simulink model "reduce_emf_simple"  (R2024b)
settings: Solver=FixedStepAuto  StartTime=0.0  StopTime=25  FixedStep=Tsim  RelTol=1e-4  EnableMultiTasking=on
InitFcn:
  | clc;
  | clear;
  | %% Parameters of the motor
  | Tsim = 1e-6;
  | Tpwm=1e-4;
  | Ts = 1e-4;
  | R = 1.8665;
  | Rs=1.8665;
  | Ls=8.96e-3;
  | Ld = 8.96e-3;
  | Lq = 8.96e-3;
  | L1=(Ld +Lq )/2;
  | L2=(Lq -Ld )/2;
  | flux = 0.21;
  | F=0.00008;
  | J=0.003;
  | Np=4;
  | fpwm = 10e3;
  | Vdc=311;
  | wn=100;
  | %% Controller limiter                                                           % Maximum torque (Nm)
  | I_max = 7.5;                                                    % Maximum current (A)
  | V_max = Vdc/sqrt(3);
  | 
  | 
  | %% 转速环电流环带宽
  | wspd=20;
  | wcur=500;
  | 
  | %% LESO
  | w0=10000;
  | beta1=2*w0-R/Ld;
  | beta2=w0*w0;
  | %% IF启动
  | Iq_if=7;
  | we_if_acc=300;
  | we_if_max=180;
  | we_switch=150;
model workspace (MAT data in the model file):
  new = 0
undefined symbols (not defined in the file or in its folder): DiscIntNeverNeededParam
libraries: spsDCVoltageSourceLib x1, spsGroundLib x1, spsPermanentMagnetSynchronousMachineLib x1, spsUniversalBridgeLib x1, spspowerguiLib x1, simulink x1
(part 2 of 2)

== matlab function reduce_emf_simple/参数辨识与采集/参数辨识算法/参数辨识 ==
  settings: updateMethod=DISCRETE  sampleTime=1e-4
  data: ud input; uq input; id input; iq input; we input; stage input; Ls output size=1; psi output size=1; Rs output size=1; da output size=1; db output size=1; doneL output size=1; doneR output size=1; run output size=1; n output size=1; ack output size=1; R0 output size=1; V0 output size=1
function [Ls, psi, Rs, da, db, doneL, doneR, run, n, ack, R0, V0] = ...
    fcn(ud, uq, id, iq, we, stage)
%#codegen
% ud、uq：V；id、iq：A；we：电角速度rad/s；采样周期Ts=100us。
% Ls：H；psi：Wb；Rs：欧姆；da、db：两组位置误差rad。
% stage=2/3/4为A组基准/正注入/负注入，6/7/8为B组，9为计算。
% run=0等待，1采样，2计算角度，3递推，30完成；负数表示数据缺失。
% n为实际递推次数，ack为采样完成的阶段号；未计算的参数为NaN。
stage = double(stage);

% 六段数据均按[ud uq id iq we]存储，每段取最后2000拍。
persistent dq_data dq_mean ready stage_z tick stopped
% 一电周期滑动平均。
persistent dq_buf dq_sum pos count N
% 跨阶段连续积分，用于修正角度计算中的电阻和逆变器压降。
persistent theta we_z ab_z int_ab int_data has_prev
% 正负注入差：电压/转速、电流/转速、电流、压降系数/转速。
persistent dU dU_w dI_w dI dV_w H F pre
% 辨识结果及RLS状态。x=[Ls/0.01; psi/0.2]仅做数值尺度归一化。
persistent L flux R delta done status ack_z loss x P it

%% 1. 初始化与阶段切换
if isempty(stage_z)
    stage_z = -1;
end
if isempty(dq_data) || ((stage == 0 || stage == 2) && stage ~= stage_z)
    dq_data = zeros(2000, 5, 6);
    dq_mean = zeros(6, 5);
    ready = false(6, 1);
    stopped = false;
    tick = 0;
    dq_buf = zeros(1257, 5);
    dq_sum = zeros(1, 5);
    pos = 0;
    count = 0;
    N = 1;
    theta = 0;
    we_z = 0;
    ab_z = zeros(1, 6);
    int_ab = zeros(1, 6);
    int_data = zeros(2000, 8, 2);
    has_prev = false;
    dU = zeros(2, 2);
    dU_w = zeros(2, 2);
    dI_w = zeros(2, 2);
    dI = zeros(2, 2);
    dV_w = zeros(2, 2);
    H = zeros(3, 3, 2);
    F = zeros(3, 6, 2);
    pre = 0;
    L = NaN;
    flux = NaN;
    R = NaN;
    delta = zeros(2, 1);
    done = zeros(2, 1);
    status = 0;
    ack_z = 0;
    loss = [NaN; NaN];
    x = zeros(2, 1);
    P = 10*eye(2);
    it = 0;
end

dq = [ud uq id iq we];
valid = all(isfinite(dq)) && isfinite(stage);
if valid && stage ~= stage_z
    stage_z = stage;
    tick = 0;
    ack_z = 0;
    dq_buf(:) = 0;
    dq_sum(:) = 0;
    pos = 0;
    count = 0;
    N = 1;
end

if ~valid
    % 非有限输入才中止；不按纹波大小或参数正负拒绝结果。
    L = NaN;
    flux = NaN;
    R = NaN;
    delta(:) = 0;
    done(:) = 0;
    loss(:) = NaN;
    ready(:) = false;
    it = 0;
    status = -1;
    ack_z = 0;
    if stage >= 2 && stage <= 8
        ack_z = -double(stage);
    end
    stopped = true;
end

%% 2. 采样：先等待0.4秒，再保存0.2秒
if ~stopped && stage >= 2 && stage <= 8
    % 积分使用外部50Hz低通后的dq量，阶段5也连续积分。
    % 它只用于压降修正，不改变控制环角度或转速。
    if has_prev
        theta = mod(theta + 0.5e-4*(we_z + we), 2*pi);
    end
    c = cos(theta);
    s = sin(theta);
    ab = [ud*c-uq*s, ud*s+uq*c, id*c-iq*s, id*s+iq*c];
    D = (4/pi)*ab(3:4)/max(hypot(id, iq), 1e-12);
    ab_now = [ab D];
    if has_prev
        int_ab = int_ab + 0.5e-4*(ab_z + ab_now);
    end
    ab_z = ab_now;
    we_z = we;
    has_prev = true;

    % A组对应存储段1~3，B组对应存储段4~6，阶段5留给恢复。
    seg = 0;
    if stage >= 2 && stage <= 4
        seg = double(stage) - 1;
    elseif stage >= 6 && stage <= 8
        seg = double(stage) - 2;
    end

    if seg > 0 && ~ready(seg)
        status = 1;
        tick = tick + 1;
        % 0.1秒时锁定周期点数；五路量使用完全相同的平均器。
        if tick == 1000
            N = min(1257, max(50, round(2*pi/(max(abs(we), 50)*1e-4))));
            dq_buf(:) = 0;
            dq_sum(:) = 0;
            pos = 0;
            count = 0;
        end
        dq_avg = dq;
        if tick >= 1000
            pos = mod(pos, N) + 1;
            dq_sum = dq_sum + dq - dq_buf(pos, :);
            dq_buf(pos, :) = dq;
            count = min(N, count + 1);
            dq_avg = dq_sum/count;
        end
        if tick > 4000 && tick <= 6000
            k = tick - 4000;
            dq_data(k, :, seg) = dq_avg;
            if seg == 1 || seg == 4
                g = 1 + (seg == 4);
                int_data(k, :, g) = [int_ab c s];
            end
        end
        if tick == 6000
            dq_mean(seg, :) = sum(dq_data(:, :, seg), 1)/2000;
            ready(seg) = true;
            ack_z = double(stage);
        end
    end
end

%% 3. 正负注入求角度，两组数据交替做参数递推
if ~stopped && stage == 9
    if ~all(ready)
        status = -2;
        stopped = true;
    elseif status == 1
        status = 2;
    elseif pre < 400
        % 每拍处理5个新样本；400拍处理完每组2000个注入样本。
        pre = pre + 1;
        for g = 1:2
            seg = 2 + 3*(g-1);
            for k = (pre-1)*5+1:pre*5
                dq_p = dq_data(k, :, seg);
                dq_m = dq_data(k, :, seg+1);
                wp = speed_safe(dq_p(5));
                wm = speed_safe(dq_m(5));
                Dp = (4/pi)*dq_p(3:4)/max(hypot(dq_p(3), dq_p(4)), 1e-12);
                Dm = (4/pi)*dq_m(3:4)/max(hypot(dq_m(3), dq_m(4)), 1e-12);
                dU(g, :) = dU(g, :) + dq_p(1:2) - dq_m(1:2);
                dU_w(g, :) = dU_w(g, :) + (dq_p(1:2)/wp - dq_m(1:2)/wm);
                dI_w(g, :) = dI_w(g, :) + (dq_p(3:4)/wp - dq_m(3:4)/wm);
                dI(g, :) = dI(g, :) + (dq_p(3:4) - dq_m(3:4));
                dV_w(g, :) = dV_w(g, :) + (Dp/wp - Dm/wm);
                h = [1; int_data(k, 7, g); int_data(k, 8, g)];
                H(:, :, g) = H(:, :, g) + h*h';
                F(:, :, g) = F(:, :, g) + h*int_data(k, 1:6, g);
            end
            delta(g) = angle_wrap(atan2(dU(g, 2), dU(g, 1)));
        end
        if pre == 400
            loss = loss_fit(H, F);
            for g = 1:2
                delta(g) = angle_fix(dU_w(g, :), dI_w(g, :), ...
                    dI(g, :), dV_w(g, :), loss, 0);
            end
        end
    else
        % A1、B1、A2、B2……每拍读取一个未使用的基准样本。
        it = it + 1;
        for g = 1:2
            delta(g) = angle_fix(dU_w(g, :), dI_w(g, :), ...
                dI(g, :), dV_w(g, :), loss, 0.01*x(1));
        end
        g = 1 + mod(it-1, 2);
        k = floor((it-1)/2) + 1;
        seg = 1 + 3*(g-1);
        ud_k = dq_data(k, 1, seg);
        uq_k = dq_data(k, 2, seg);
        id_k = dq_data(k, 3, seg);
        iq_k = dq_data(k, 4, seg);
        we_k = dq_data(k, 5, seg);

        % 稳态方程消去R：uq*id-ud*iq = we*Ls*(id²+iq²)
        %                                 + we*psi*(id*cos(delta)+iq*sin(delta))。
        phi = [0.01*we_k*(id_k^2+iq_k^2); ...
            0.2*we_k*(id_k*cos(delta(g))+iq_k*sin(delta(g)))];
        scale = max(norm(phi), 1e-12);
        phi = phi/scale;
        u = (uq_k*id_k - ud_k*iq_k)/scale;
        K = P*phi/(1 + phi'*P*phi);
        e = u - phi'*x;
        x = x + K*e;
        % Joseph形式更新协方差，遗忘因子为1。
        A = eye(2) - K*phi';
        P = A*P*A' + K*K';
        P = 0.5*(P + P');
        L = 0.01*x(1);
        flux = 0.2*x(2);
        R = rs_calc(dq_mean, delta, L, flux);
        status = 3;
        if it == 4000
            done(1) = double(all(isfinite(x)));
            done(2) = double(isfinite(R));
            status = 30;
            stopped = true;
        end
    end
end

if ~stopped && stage == 10
    status = -10;
    stopped = true;
end

%% 4. 各电气量独立输出
Ls = L;
psi = flux;
Rs = R;
da = delta(1);
db = delta(2);
doneL = done(1);
doneR = done(2);
run = status;
n = it;
ack = ack_z;
R0 = loss(1);
V0 = loss(2);
end

function a = angle_fix(dU_w, dI_w, dI, dV_w, loss, Ls)
% 正负注入的ud/we、uq/we差分；修正电阻、压降和电流变化的影响。
% R0、V0来自数据标定，Ls来自当前RLS结果，不预填额定参数。
fd = dU_w(1) - loss(1)*dI_w(1) + Ls*dI(2) - loss(2)*dV_w(1);
fq = dU_w(2) - loss(1)*dI_w(2) - Ls*dI(1) - loss(2)*dV_w(2);
a = angle_wrap(atan2(fq, fd));
end

function a = angle_wrap(a)
% 位置误差取论文反正切对应的[-pi/2, pi/2]分支。
if a > pi/2
    a = a - pi;
elseif a < -pi/2
    a = a + pi;
end
end

function loss = loss_fit(H, F)
% 压降修正的辅助计算，不是论文的主参数RLS。
% 将积分量拟合为常值+余弦+正弦，取两个工作点的积分中心差。
% 静止坐标系电压方程给出：DeltaU = R0*DeltaI + V0*DeltaD。
center = zeros(2, 6);
for g = 1:2
    coef = (H(:, :, g) + 1e-10*eye(3))\F(:, :, g);
    center(g, :) = coef(1, :);
end
dInt = center(2, :) - center(1, :);
B = [dInt(3:4)', dInt(5:6)'];
u = dInt(1:2)';
scale = max(sqrt(sum(sum(B.^2))), 1e-12);
B = B/scale;
u = u/scale;
loss = (B'*B + 1e-10*eye(2))\(B'*u);
end

function Rs = rs_calc(dq_mean, delta, Ls, psi)
% 两组q轴方程：uq-we*Ls*id-we*psi*cos(delta) = Rs*iq + V0*Dq。
% 消去共同的V0，每次使用新Ls、psi更新Rs；不直接复制辅助电阻R0。
Dq = zeros(2, 1);
uq_res = zeros(2, 1);
for g = 1:2
    seg = 1 + 3*(g-1);
    id = dq_mean(seg, 3);
    iq = dq_mean(seg, 4);
    we = dq_mean(seg, 5);
    Dq(g) = (4/pi)*iq/max(hypot(id, iq), 1e-8);
    uq_res(g) = dq_mean(seg, 2) - we*Ls*id - we*psi*cos(delta(g));
end
den = Dq(2)*dq_mean(1, 4) - Dq(1)*dq_mean(4, 4);
scale = abs(Dq(2)*dq_mean(1, 4)) + abs(Dq(1)*dq_mean(4, 4));
if abs(den) > 64*eps(max(scale, 1))
    Rs = (Dq(2)*uq_res(1) - Dq(1)*uq_res(2))/den;
else
    Rs = NaN;
end
end

function we = speed_safe(we)
% 只避免浮点除零，不设置转速验收门限。
if abs(we) < 1e-9
    if we < 0
        we = -1e-9;
    else
        we = 1e-9;
    end
end
end

== matlab function reduce_emf_simple/电流采样与矢量控制/SVPWM/SVPWM/N Caculate/MATLAB Function ==
  data: u input; y output
function y = fcn(u)
if u==0
    y=1;
else
    y = u;
end

== matlab function reduce_emf_simple/MATLAB Function2 ==
  data: n input; n_filt output
function n_filt = fcn(n)
%#codegen
% 五路共用相同的50 Hz低通；周期平均在参数辨识函数内部执行。
n_filt=n;
end

== matlab function reduce_emf_simple/反电动势观测与锁相环/MATLAB Function1 ==
  data: n input; n_filt output
function n_filt = fcn(n)
%#codegen
% 文档图12.2的PLL速度反馈接口；输入来自原有一拍延迟的PLL速度。
% 本版旁路原100Hz低通，确保角度推进与解耦使用同一拍速度。
n_filt = n;
end

== matlab function reduce_emf_simple/备用模型_已停用/Subsystem/MATLAB Function1 ==
  data: u input; y output; deta input
function y = fcn(u,deta)
a=1e-6;
if u<a
    y=0;
else
    y=deta;
end

== matlab function reduce_emf_simple/反电动势观测与锁相环/锁相环1/MATLAB Function ==
  settings: updateMethod=DISCRETE  sampleTime=1e-4
  data: Ed_hat input size=1; Eq_hat input size=1; theta output size=1; we output size=1; IF_sensorless_mode input; id_offset output; vfl_state output; sample_ack input
function [theta,we,id_offset,vfl_state] = fcn(Ed_hat,Eq_hat,IF_sensorless_mode,sample_ack)
%#codegen
%==================================================
% 文档式(12.7)、图12.2：反电动势相位误差 -> PI -> 角度积分。
% Ed_hat、eb端口现在分别接Ed_hat、Eq_hat，单位V，不再接磁链。
% 虚拟反电动势注入与六段采样；Id切入退出用100毫秒斜坡。
% 保留原有I/F切换输入及四路输出，外围控制连接保持完整。
%==================================================
persistent theta_z speed_i state tick stable amp id_ramp
if isempty(theta_z)
    theta_z = 0;
    speed_i = 0;
    state=0; tick=0; stable=0; amp=0; id_ramp=0;
end
if ~isfinite(Ed_hat) || ~isfinite(Eq_hat) || ~isfinite(IF_sensorless_mode)
    Ed_hat=0; Eq_hat=0; IF_sensorless_mode=0;
end
Ts = 1e-4;                    % 原控制周期，s
wn = 50;                      % PLL带宽初值，rad/s；沿用原代码数值
kp = 2*0.707*wn;              % PI比例增益
ki = wn*wn;                   % PI积分增益
we_max = 1256;                % 原电角速度限幅，rad/s
E_min = 1e-3;                 % 反电动势不足时不更新相位误差，V

% 状态输出与采集函数共用同一控制周期；1表示已切换至无感控制。
% 虚拟电压仅加到PLL使用的Ed，不直接叠加到电机电压命令。
id_offset=0; injection=0;
if IF_sensorless_mode<0.5 || ~isfinite(Ed_hat+Eq_hat)
    state=0; tick=0; stable=0;
end
if state>0
    tick=tick+1;
    % 调试版每个采样阶段固定0.6秒；不等待稳态、工作点或条件数验收。
    % 确认口只保留非有限输入时的数值错误中止，不接受质量门限中止。
    if state>=2 && state<=8 && sample_ack<0
        state=10; tick=0;
    % 工作点切换共1秒，包含100毫秒Id斜坡和900毫秒恢复时间。
    elseif state==5 && tick>10000
        state=6; tick=1;
        amp=min(0.6,max(0.2,0.01*abs(Eq_hat)));
    elseif state>=2 && state<=8 && state~=5 && tick>6000
        state=state+1; tick=1;
    end
    if state>=5 && state<=8, id_offset=-1.0; end
    if state==3 || state==7, injection=amp;
    elseif state==4 || state==8, injection=-amp;
    end
end
% 正常实验时Id偏移按10 A/s变化，沿用100微秒控制周期。
% I/F复位或数值错误中止时立即清零，不延迟原有复位动作。
if IF_sensorless_mode<0.5 || state==10
    id_ramp=0;
else
    id_step=10*Ts;
    id_ramp=id_ramp+min(max(id_offset-id_ramp,-id_step),id_step);
end
% 仅在恢复段内加入200毫安的平滑标定激励，用于分离电阻与逆变器压降。
% 150～350毫秒启用，之后仍有650毫秒恢复；六个正式采样段不加此激励。
id_calibration=0;
if state==5 && tick>=1500 && tick<=3500
    pulse_time=(tick-1500)*Ts;
    envelope=sin(pi*pulse_time/0.2)^2;
    id_calibration=0.2*envelope*cos(theta_z);
end
id_offset=id_ramp+id_calibration;
vfl_state=int32(state);
Ed_pll=Ed_hat+injection;

% 文档式(12.7)，严格保留atan比值的正负转速语义。
% 分母正则化只用于避免Eq=0数值除零，不改为磁链q轴误差。
if Ed_hat*Ed_hat+Eq_hat*Eq_hat>E_min*E_min
    eq_safe = Eq_hat;
    if abs(eq_safe)<1e-6
        if eq_safe>=0
            eq_safe = 1e-6;
        else
            eq_safe = -1e-6;
        end
    end
    phase_error = atan(-Ed_pll/eq_safe);
else
    phase_error = 0;
end

% PI输出电角速度；限幅饱和时采用条件积分抑制积分累积。
we_unsat = speed_i+kp*phase_error;
we = min(max(we_unsat,-we_max),we_max);
if (we_unsat<=we_max && we_unsat>=-we_max) || ...
   (we_unsat>we_max && phase_error<0) || ...
   (we_unsat< -we_max && phase_error>0)
    speed_i = speed_i+ki*Ts*phase_error;
end
speed_i = min(max(speed_i,-we_max),we_max);

% 输出本周期角度，再以同周期速度推进下一拍角度。
% 外部一拍角度反馈和一拍速度反馈，避免代数环并保持采样对齐。
theta = theta_z;
theta_z = mod(theta_z+Ts*we,2*pi);
% 原有I/F切换至无感0.5秒后开始实验，不再增加相位、速度趋势验收。
% 此处触发的状态转换从下一拍输出，保持注入与状态标记一致。
if state==0 && IF_sensorless_mode>=0.5
    stable=stable+1;
    if stable>=5000
        state=2; tick=0; stable=0;
        amp=min(0.6,max(0.2,0.01*abs(Eq_hat)));
    end
elseif state==0
    stable=0;
end
% 状态9计算结果并将Id偏移斜坡恢复为0；状态10立即中止并清零。
end

== matlab function reduce_emf_simple/反电动势观测与锁相环/反电动势观测器 ==
  data: ua input; Ed_hat output; ub input; ia input; ib input; Eq_hat output; we input; theta_hat output; we_out output; theta_z1 input
function [Ed_hat,Eq_hat,theta_hat,we_out] = fcn_improved_paper_strict(ua,ub,ia,ib,we,theta_z1)
%#codegen
%==================================================
% 文档式(12.5)、(12.6)及图12.2：dq降阶扩展反电动势观测器。
% 当前对象为SPMSM，Ld=Lq=Ls，扩展反电动势即永磁体反电动势。
% 输入ua/ub、ia/ib为alpha-beta电压和电流，we为延迟一拍的PLL电角速度。
% theta_z1为延迟一拍的PLL角度，先按同一拍we推进至当前时刻。
% 输出Ed_hat/Eq_hat单位V，直接送入反电动势PLL，不再转换成磁链。
%==================================================
persistent zd zq bd_old bq_old
Ts = 1e-4;                    % 原模型控制周期，s
Ls = 8.96e-3;                 % 参考电感，H
Rs = 1.8665;                  % 参考电阻，ohm
Gr = 500;                     % 所选观测器增益初值，rad/s；文档未给定数值

% 将延迟角度推进一拍，与本周期电压、电流对齐。
theta_c = mod(theta_z1+Ts*we,2*pi);
cs = cos(theta_c);
sn = sin(theta_c);
ud =  cs*ua+sn*ub;
uq = -sn*ua+cs*ub;
id =  cs*ia+sn*ib;
iq = -sn*ia+cs*ib;

% 文档式(12.6)的解耦电压。
ud1 = ud+we*Ls*iq;
uq1 = uq-we*Ls*id;

% 图12.2的降阶实现：
% E_hat = Gr/(s+Gr) * (u_dq1-Rs*i_dq-Ls*p*i_dq)。
% 定义z=E_hat+Gr*Ls*i，消除显式电流微分：
% z_dot=-Gr*z+Gr*(u_dq1+(Gr*Ls-Rs)*i_dq)。
% 两个轴独立，采用梯形法离散，保持100us控制周期。
bd = Gr*(ud1+(Gr*Ls-Rs)*id);
bq = Gr*(uq1+(Gr*Ls-Rs)*iq);
if isempty(zd)
    zd = Gr*Ls*id;            % 初始Ed_hat=0
    zq = Gr*Ls*iq;            % 初始Eq_hat=0
    bd_old = bd;
    bq_old = bq;
else
    a = 0.5*Ts*Gr;
    zd = ((1-a)*zd+0.5*Ts*(bd+bd_old))/(1+a);
    zq = ((1-a)*zq+0.5*Ts*(bq+bq_old))/(1+a);
    bd_old = bd;
    bq_old = bq;
end
Ed_hat = zd-Gr*Ls*id;
Eq_hat = zq-Gr*Ls*iq;

% 辅助监测输出，主闭环只使用前两路反电动势。
if abs(Ed_hat)+abs(Eq_hat)>1e-6
    eq_safe = Eq_hat;
    if abs(eq_safe)<1e-6
        if eq_safe>=0
            eq_safe=1e-6;
        else
            eq_safe=-1e-6;
        end
    end
    theta_hat = mod(theta_c+atan(-Ed_hat/eq_safe),2*pi);
else
    theta_hat = theta_c;
end
we_out = we;
end
